simulink library "Disabled_lib"  (R2023b)
settings: Solver=VariableStepAuto  StartTime=0.0  StopTime=10.0  RelTol=1e-3
undefined symbols (not defined in the file): Spline_Num_Poses_default, Spline_Ref_Poses_default
settings Model: Creator=FIRSTMentor  LastModifiedBy=ander

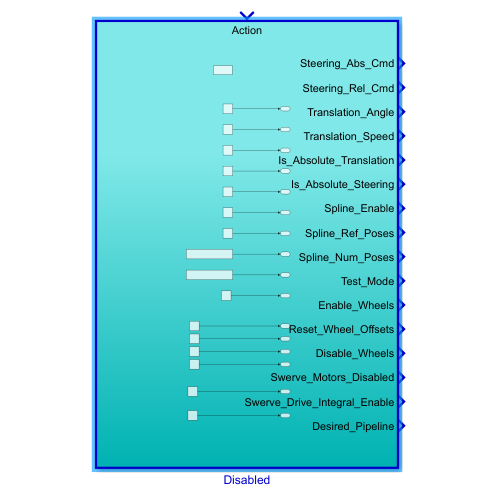
[thumbnail: Simulink's stored preview of the top-level diagram]
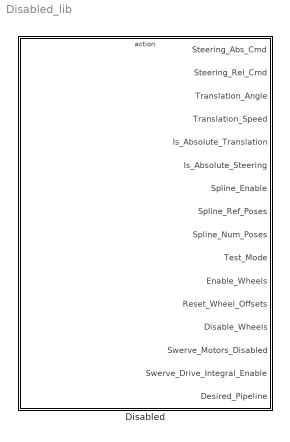
== system Disabled_lib ==
  Disabled : Subsystem  TreatAsAtomicUnit=on

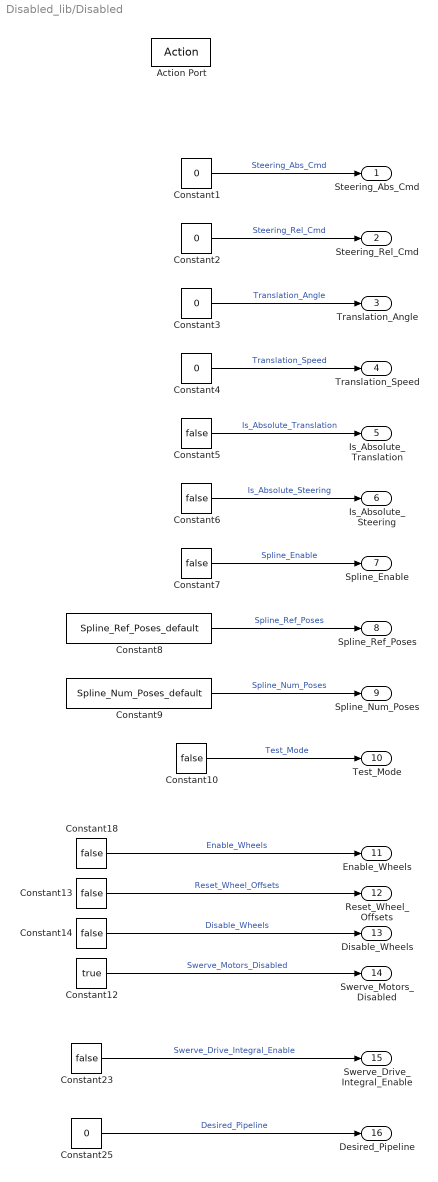
== system Disabled_lib/Disabled ==
  Action Port : ActionPort
  Constant{1..4} (4 alike) : Constant  Value=0
  Constant{7,10,13..14,18,23} (6 alike) : Constant  Value=false  OutDataTypeStr=boolean
  Constant12 : Constant  Value=true  OutDataTypeStr=boolean
  Constant25 : Constant  Value=0  OutDataTypeStr=uint8
  Constant5 : Constant  Value=false
  Constant6 : Constant  Value=false
  Constant8 : Constant  Value=Spline_Ref_Poses_default
  Constant9 : Constant  Value=Spline_Num_Poses_default  OutDataTypeStr=double
  Steering_Abs_Cmd : Outport
  Steering_Rel_Cmd : Outport  Port=2
  Translation_Angle : Outport  Port=3
  Translation_Speed : Outport  Port=4
  Is_Absolute_Translation : Outport  Port=5
  Is_Absolute_Steering : Outport  Port=6
  Spline_Enable : Outport  Port=7
  Spline_Ref_Poses : Outport  Port=8
  Spline_Num_Poses : Outport  Port=9
  Test_Mode : Outport  Port=10
  Enable_Wheels : Outport  Port=11
  Reset_Wheel_Offsets : Outport  Port=12
  Disable_Wheels : Outport  Port=13
  Swerve_Motors_Disabled : Outport  Port=14
  Swerve_Drive_Integral_Enable : Outport  Port=15
  Desired_Pipeline : Outport  Port=16
  wires:
  Constant1/1 -> Steering_Abs_Cmd/1  "Steering_Abs_Cmd"
  Constant2/1 -> Steering_Rel_Cmd/1  "Steering_Rel_Cmd"
  Constant3/1 -> Translation_Angle/1  "Translation_Angle"
  Constant4/1 -> Translation_Speed/1  "Translation_Speed"
  Constant5/1 -> Is_Absolute_Translation/1  "Is_Absolute_Translation"
  Constant6/1 -> Is_Absolute_Steering/1  "Is_Absolute_Steering"
  Constant7/1 -> Spline_Enable/1  "Spline_Enable"
  Constant8/1 -> Spline_Ref_Poses/1  "Spline_Ref_Poses"
  Constant9/1 -> Spline_Num_Poses/1  "Spline_Num_Poses"
  Constant10/1 -> Test_Mode/1  "Test_Mode"
  Constant14/1 -> Disable_Wheels/1  "Disable_Wheels"
  Constant13/1 -> Reset_Wheel_Offsets/1  "Reset_Wheel_Offsets"
  Constant12/1 -> Swerve_Motors_Disabled/1  "Swerve_Motors_Disabled"
  Constant18/1 -> Enable_Wheels/1  "Enable_Wheels"
  Constant23/1 -> Swerve_Drive_Integral_Enable/1  "Swerve_Drive_Integral_Enable"
  Constant25/1 -> Desired_Pipeline/1  "Desired_Pipeline"
